simulink model "Ah_Integrator_Estimator"  (R2025b)
settings: Solver=FixedStepDiscrete  StartTime=0.0  StopTime=10.0  FixedStep=0.1  RelTol=1e-3
values from neighbouring files (symbols this model uses):
  eta_coulomb = 0.99    [Ah_Integrator_Estimator.sldd]
  Q_rated = 1200.0    [Ah_Integrator_Estimator.sldd]
undefined symbols (not defined in the file or in its folder): DiscIntNeverNeededParam
settings Model: DataDictionary=Ah_Integrator_Estimator.sldd  Creator=admin  LastModifiedBy=admin
settings OptimizationCC: DefaultParameterBehavior=Inlined  EnhancedBackFolding=on  PassReuseOutputArgsAs=Individual arguments  ActiveStateOutputEnumStorageType=uint8  ZeroExternalMemoryAtStartup=off  ZeroInternalMemoryAtStartup=off  EfficientFloat2IntCast=on  OptimizeBlockOrder=speed  DifferentSizesBufferReuse=on  OptimizationCustomize=off  EfficientTunableParamExpr=on
settings DebuggingCC: ParameterTunabilityLossMsg=error
settings HardwareCC: ProdBitPerPointer=32.0  ProdBitPerSizeT=32.0  ProdBitPerPtrDiffT=32.0  ProdLargestAtomicInteger=Long  ProdLargestAtomicFloat=Double  ProdWordSize=32.0  ProdHWDeviceType=ARM Compatible->ARM Cortex-M
settings SFSimCC: MATLABDynamicMemAlloc=off
settings RTWCC: SystemTargetFile=ert.tlc  GenCodeOnly=on  TemplateMakefile=ert_default_tmf  GenerateReport=on  IncludeHyperlinkInReport=on  LaunchReport=on  GenerateTraceInfo=on  GenerateTraceReportSl=on  GenerateTraceReportSf=on  GenerateWebview=on  GPUComputeCapability=3.5  Description=Embedded Coder
settings CodeAppCC: ForceParamTrailComments=on  IgnoreCustomStorageClasses=off  OperatorAnnotations=on  SimulinkDataObjDesc=on  SFDataObjDesc=on  InsertBlockDesc=on
settings ERTTargetCC: ERTCustomFileTemplate=example_file_process.tlc  ERTFilePackagingFormat=CompactWithDataFile  DynamicArrayContainerType=coder::array  TargetLangStandard=C99 (ISO)  IncludeMdlTerminateFcn=off  SupportNonFinite=off  SupportComplex=off  RemoveDisableFunc=on

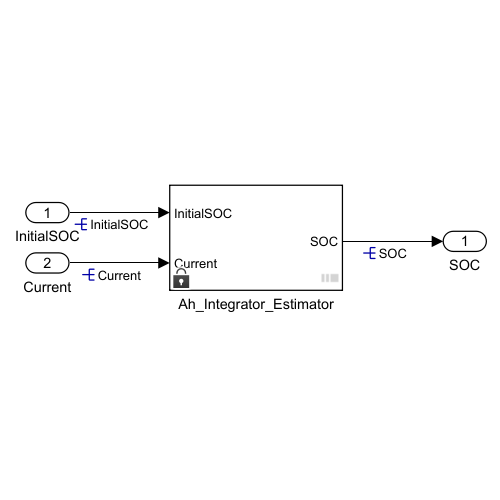
[thumbnail: Simulink's stored preview of the top-level diagram]
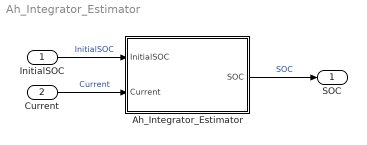
== system Ah_Integrator_Estimator ==
  InitialSOC : Inport
  Current : Inport  Port=2
  Ah_Integrator_Estimator : Subsystem
  SOC : Outport
  wires:
  InitialSOC/1 -> Ah_Integrator_Estimator/1(InitialSOC)  "InitialSOC"
  Current/1 -> Ah_Integrator_Estimator/2(Current)  "Current"
  Ah_Integrator_Estimator/1(SOC) -> SOC/1  "SOC"

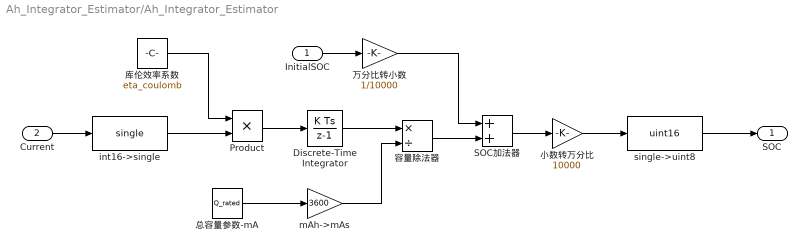
== system Ah_Integrator_Estimator/Ah_Integrator_Estimator ==
  InitialSOC : Inport
  Current : Inport  Port=2
  Discrete-Time Integrator : DiscreteIntegrator  SampleTime=-1  ICPrevOutput=DiscIntNeverNeededParam  ICPrevScaledInput=DiscIntNeverNeededParam
  Product : Product
  SOC加法器 : Sum
  int16->single : DataTypeConversion  OutDataTypeStr=single  SaturateOnIntegerOverflow=off  RndMeth=Floor
  mAh->mAs : Gain  Gain=3600  OutDataTypeStr=single
  single->uint8 : DataTypeConversion  OutDataTypeStr=uint16  RndMeth=Round
  万分比转小数 : Gain  Gain=1/10000  OutDataTypeStr=single
  容量除法器 : Product  Inputs=*/
  小数转万分比 : Gain  Gain=10000
  库伦效率系数 : Constant  Value=eta_coulomb  LockScale=on
  总容量参数-mA : Constant  Value=Q_rated  LockScale=on
  SOC : Outport
  wires:
  容量除法器/1 -> SOC加法器/2
  mAh->mAs/1 -> 容量除法器/2
  Discrete-Time Integrator/1 -> 容量除法器/1
  SOC加法器/1 -> 小数转万分比/1
  总容量参数-mA/1 -> mAh->mAs/1
  库伦效率系数/1 -> Product/1
  Current/1 -> int16->single/1
  Product/1 -> Discrete-Time Integrator/1
  single->uint8/1 -> SOC/1
  int16->single/1 -> Product/2
  小数转万分比/1 -> single->uint8/1
  InitialSOC/1 -> 万分比转小数/1
  万分比转小数/1 -> SOC加法器/1
